simulink library "casper_library_correlator"  (Simulink 8.0)
settings: Solver=ode45  SolverMode=SingleTasking  StartTime=0.0  StopTime=10.0  RelTol=1e-3
values from neighbouring files (symbols this model uses):
  n_bits = eval(get_var('n_bits', 'defaults', defaults, varargin{:}))    [auto_tap_init.m]    (also in baseline_tap_init.m; bi_real_unscr_2x_init.m = get_var('n_bits', 'defaults', defaults, varargin{:}); bi_real_unscr_4x_init.m = get_var('n_bits', 'defaults', defaults, varargin{:}); bit_reverse_init.m = get_var('n_bits',varargin{:}))
libraries: xbsIndex_r4 x1360, casper_library_misc x140, casper_library_multipliers x32, xps_library x8, casper_library_delays x1, casper_library_correlator x1
(part 1 of 14)
settings Model: Creator=mdexter  LastModifiedBy=jmanley

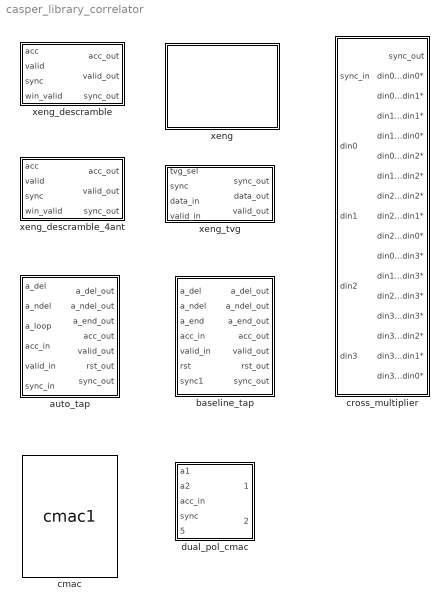
== system casper_library_correlator ==
  auto_tap : Subsystem  mask(auto_tap){n_ants=4, n_simultan=2, n_bits=4, acc_len=64, add_latency=1, mult_latency=2, bram_latency=2, mult_type=0, use_bram_delay=1}
      mask prompts: n_ants "Number of antennas (total inputs = n_ants*n_simultan below)"; n_simultan "Number of inputs fed-in simultaneously"; n_bits "Number of input bits (per complex component)"; acc_len "Accumulation length"; add_latency "Adder latency"; mult_latency "Multiplier latency"; bram_latency "BRAM latency"; mult_type "Multiplier Type (0=behavioural HDL, 1=embedded, 2=core)"; use_bram_delay "Implementation: Delay type (0=SLR, 1=BRAM)"
      mask init:
      | fix_pnt_pos = (n_bits-1)*2;
      | bit_growth = ceil(log2(acc_len));
      | ant_bits = ceil(log2(n_ants));
      | n_bits_out = (2*n_bits + 1 + bit_growth);
      | 
      | params = get_mask_params(gcb);
      | auto_tap_init(gcb, params{:});
      settings: AttributesFormatString=mult_typ=0, del_typ=1
  baseline_tap : Subsystem  mask(baseline_tap){n_ants=4, ant_sep=1, n_bits=4, acc_len=32, add_latency=1, mult_latency=2, bram_latency=2, mult_type=2, use_bram_delay=1}
      mask prompts: n_ants "Number of antennas"; ant_sep "Antenna Seperation"; n_bits "number of input bits (per complex component)"; acc_len "accumulation length"; add_latency "Adder latency"; mult_latency "Multiplier latency"; bram_latency "BRAM latency"; mult_type "Multiplier Type (0=behavioural HDL, 1=embedded, 2=core)"; use_bram_delay "Use BRAM delays"
      mask init:
      | fix_pnt_pos = (n_bits-1)*2;
      | bit_growth = ceil(log2(acc_len));
      | ant_bits = ceil(log2(n_ants));
      | n_bits_out = (2*n_bits + 1 + bit_growth);
      | 
      | params = get_mask_params(gcb);
      | baseline_tap_init(gcb, params{:});
      settings: AttributesFormatString=ant_sep=1, mult=2, bram=1
  cmac : casper_library_correlator/dual_pol_cmac/cmac1  Tag=cmac  acc_len=128  n_bits_a=4  bin_pt_a=3  n_bits_b=4  bin_pt_b=3  quantization=Truncate  overflow=Wrap  mult_latency=1  add_latency=1  in_latency=0  conv_latency=0  multiplier_implementation=embedded multiplier core
  cross_multiplier : Subsystem  mask(cross_multiplier){streams=4, aggregation=2, bit_width_in=4, binary_point_in=3, bit_width_out=9, binary_point_out=6, mult_latency=2, add_latency=1, overflow=Wrap, quantisation=Truncate, conv_latency=0}
      mask prompts: streams "Number input streams"; aggregation "Aggregation per stream"; bit_width_in "Bit width in"; binary_point_in "Binary point in"; bit_width_out "Bit width out"; binary_point_out "Binary point out"; mult_latency "Multiplier latency"; add_latency "Adder latency"; overflow "Overflow behaviour"; quantisation "Quantisation behaviour"; conv_latency "Bit width conversion latency"
      mask help: Cross multiplies aggregated complex input streams.
      mask init:
      | cross_multiplier_init(gcb, ...
      |     'streams', streams, ...
      |     'aggregation', aggregation, ...
      |     'bit_width_in', bit_width_in, ...
      |     'binary_point_in', binary_point_in, ...
      |     'bit_width_out', bit_width_out, ...
      |     'binary_point_out', binary_point_out, ...
      |     'mult_latency', mult_latency, ...
      |     'add_latency', add_latency, ...
      |     'overflow', overflow, ...
      |     'quantisation', quantisation, ...
      |     'conv_latency', conv_latency);
      mask TypeOptions overflow: Wrap | Saturate | Error
      mask TypeOptions quantisation: Truncate | Round  (unbiased: +/- Inf) | Round  (unbiased: even values)
  dual_pol_cmac : Subsystem  AncestorBlock=casper_library_correlator/dual_pol_cmac  mask{acc_len=128, n_bits_in=4, bin_pt_in=3, mult_latency=1, add_latency=1, multiplier_implementation=embedded multiplier core}
      mask prompts: acc_len "Number of accumulations"; n_bits_in "Number of bits in"; bin_pt_in "Binary point in"; mult_latency "Multiplier latency"; add_latency "Adder latency"; multiplier_implementation "Multiplier implementation"
      mask init:
      | bit_growth = ceil(log2(acc_len));
      | n_bits_out = (n_bits_in*2 + 1 + bit_growth);
      | bin_pt_out=(bin_pt_in*2);
      | 
      | cmacs = find_system(gcb, 'lookUnderMasks', 'all', 'FollowLinks','on','tag', 'cmac');
      | for i=1:length(cmacs),
      |     reuse_block(get_param(cmacs{i},'Parent'),get_param(cmacs{i},'Name'),'casper_library_correlator/cmac',...
      |             'mult_latency',num2str(mult_latency),...            
      |             'add_latency',num2str(add_latency),...
      |             'acc_len',num2str(acc_len),...
      |             'n_bits_a',num2str(n_bits_in),...
      |             'n_bits_b',num2str(n_bits_in),...
      |             'bin_pt_a',num2str(n_bits_in-1),...
      |             'bin_pt_b',num2str(n_bits_in-1),...
      |             'multiplier_implementation',multiplier_implementation,...
      |             'LinkStatus','inactive');
      | end
      mask TypeOptions multiplier_implementation: behavioral HDL | standard core | embedded multiplier core
  xeng : Subsystem  Tag=casper:xeng  mask(xeng){n_ants=0, n_bits=4, acc_len=128, demux_factor=4, add_latency=1, mult_latency=1, bram_latency=2, use_ded_mult=1, use_bram_delay=1}
      mask prompts: n_ants "Number of antennas"; n_bits "Bit-width of samples in"; acc_len "Accumulation length"; add_latency "Adder latency"; mult_latency "Multiplier latency"; bram_latency "BRAM latency"; use_ded_mult "Implementation: Multiplier type (0=slices 1=embedded 2=bram)"; use_bram_delay "Implementation: Delay type (0=SLR, 1=BRAM)"
      mask help: CASPER X engine with added internal valid data masking functionality, descramble and integral demux. Based on Aaron Parsons' and Lynn Urry's original X engine design.
      mask init:
      | xeng_init(gcb, ...
      |     'n_ants', n_ants, ...
      |     'n_bits', n_bits, ...
      |     'acc_len', acc_len, ...
      |     'demux_factor', demux_factor, ...
      |     'add_latency', add_latency, ...
      |     'mult_latency', mult_latency, ...
      |     'bram_latency', bram_latency, ...
      |     'use_ded_mult', use_ded_mult, ...
      |     'use_bram_delay', use_bram_delay);
      mask TypeOptions demux_factor: 1 | 2 | 4 | 8
  xeng_descramble : Subsystem  mask(xeng_descramble){num_ants=8, n_bits=4, acc_len=128, demux_factor=8}
      mask prompts: num_ants "Number of Antennas"; n_bits "Input Bitwidth"; acc_len "X engine accumulation length"; demux_factor "Demux Factor"
      mask help:
      | NOT TESTED FOR non-2^N antennas.
      |
      | Descrambles X engine output. Optionally demuxes output.
      mask init:
      | num_taps = floor(num_ants/2) + 1;
      | ant_bits = ceil(log2(num_ants));
      | num_validins = num_ants*num_taps;
      | validin_bits = floor(log2(num_validins))+1;
      | demux_bits = floor(log2(demux_factor))+1;
      | acc_len_bits = floor(log2(acc_len))+1;
      | num_ants_bits = floor(log2(num_ants))+1;
      | taps_bits = floor(log2(num_taps))+1;
      | pivot_pnt = num_ants/2*(num_taps) + num_taps*num_ants/4;
      | num_elements = nchoosek(num_ants, 2) + num_ants;
      | elements_bits = floor(log2(num_elements)) + 1;
      | n_bits_xeng_out = (2*n_bits + acc_len_bits);
      | n_bits_in = 2^(ceil(log2(n_bits_xeng_out)))*8;
      | 
      | ship_el_del = floor(acc_len*num_ants/num_validins/demux_factor) - 1;
      | 
      | if (ship_el_del < 0)
      |     errordlg('Insufficient output space for this configuration. Try a lower demux setting. Else you need fewer antennas or longer xeng acc time.');
      |     ship_el_del=0;
      | end
      | 
      | if (ship_el_del == 0)
      |     ship_el_cnt = demux_factor*num_elements-1;
      |     %in this case we're outputting multiple words back-to-back.
      | else
      |     ship_el_cnt = demux_factor*num_elements;
      |     %in this case we're outputting one word at a time.
      | end
      | 
      | ship_el_del_bits = ceil(log2(ship_el_del + 1));
      | 
      | if (ship_el_del_bits == 0)
      |     ship_el_del_bits =1;
      | end
      | 
      | fmtstr = sprintf('num_ants=%d',num_ants);
      | set_param(gcb, 'AttributesFormatString', fmtstr);
      settings: AttributesFormatString=num_ants=8
  xeng_descramble_4ant : Subsystem  mask(xeng_descramble){n_bits=4, acc_len=128, demux_factor=8}
      mask prompts: n_bits "Input Bitwidth"; acc_len "X engine accumulation length"; demux_factor "Demux Factor"
      mask help:
      | NOT TESTED FOR non-2^N antennas.
      |
      | Descrambles X engine output. Optionally demuxes output.
      mask init:
      | num_ants=4;
      | num_taps = floor(num_ants/2) + 1;
      | ant_bits = ceil(log2(num_ants));
      | num_validins = num_ants*num_taps;
      | validin_bits = floor(log2(num_validins))+1;
      | demux_bits = floor(log2(demux_factor))+1;
      | acc_len_bits = floor(log2(acc_len))+1;
      | num_ants_bits = floor(log2(num_ants))+1;
      | taps_bits = floor(log2(num_taps))+1;
      | pivot_pnt = num_ants/2*(num_taps) + num_taps*num_ants/4;
      | num_elements = nchoosek(num_ants, 2) + num_ants;
      | elements_bits = floor(log2(num_elements)) + 1;
      | n_bits_xeng_out = (2*n_bits + acc_len_bits);
      | n_bits_in = 2^(ceil(log2(n_bits_xeng_out)))*8;
      | 
      | ship_el_del = floor(acc_len*num_ants/num_validins/demux_factor) - 1;
      | 
      | if (ship_el_del < 0)
      |     errordlg('Insufficient output space for this configuration. Try a lower demux setting. Else you need fewer antennas or longer xeng acc time.');
      |     ship_el_del=0;
      | end
      | 
      | if (ship_el_del == 0)
      |     ship_el_cnt = demux_factor*num_elements-1;
      |     %in this case we're outputting multiple words back-to-back.
      | else
      |     ship_el_cnt = demux_factor*num_elements;
      |     %in this case we're outputting one word at a time.
      | end
      | 
      | ship_el_del_bits = ceil(log2(ship_el_del + 1));
      | 
      | if (ship_el_del_bits == 0)
      |     ship_el_del_bits =1;
      | end
      | 
      | fmtstr = sprintf('num_ants=%d',num_ants);
      | set_param(gcb, 'AttributesFormatString', fmtstr);
      settings: AttributesFormatString=num_ants=4
  xeng_tvg : Subsystem  mask{ant_bits=2, x_int_bits=5, sync_period=15}
      mask prompts: ant_bits "Number of Antennas (2^?):"; x_int_bits "X Integration Length (2^?):"; sync_period "Sync Pulse Period (2^?):"

== system casper_library_correlator/auto_tap ==
  a_del : Inport
  a_ndel : Inport  Port=2
  a_loop : Inport  Port=3
  acc_in : Inport  Port=4
  valid_in : Inport  Port=5
  sync_in : Inport  Port=6
  delay : Subsystem  AncestorBlock=casper_library_delays/delay_bram  mask(delay_bram){DelayLen=126, bram_latency=2, use_dsp48=off, async=off}
      mask prompts: DelayLen "Delay By:"; bram_latency "BRAM Latency"; use_dsp48 "Use DSP48"; async "asynchronous operation"
      mask help: A delay block that uses BRAM for its storage.
      mask init:
      | delay_bram_init(gcb, ...
      |     'DelayLen', DelayLen, ...
      |     'bram_latency', bram_latency, ...
      |     'use_dsp48', use_dsp48, ...
      |     'async', async);
      mask Help: eval('xlWeb(''http://casper.berkeley.edu/wiki/Delay_bram'')')
  dual_pol_cmac : Subsystem  AncestorBlock=casper_library_correlator/dual_pol_cmac  mask{acc_len=128, n_bits_in=4, bin_pt_in=3, mult_latency=1, add_latency=1, multiplier_implementation=embedded multiplier core}
      mask prompts: acc_len "Number of accumulations"; n_bits_in "Number of bits in"; bin_pt_in "Binary point in"; mult_latency "Multiplier latency"; add_latency "Adder latency"; multiplier_implementation "Multiplier implementation"
      mask init: same as casper_library_correlator/dual_pol_cmac
      mask TypeOptions multiplier_implementation: behavioral HDL | standard core | embedded multiplier core
  sync_delay : casper_library_delays/sync_delay  DelayLen=71
  a_del_out : Outport
  a_ndel_out : Outport  Port=2
  a_end_out : Outport  Port=3
  acc_out : Outport  Port=4
  valid_out : Outport  Port=5
  rst_out : Outport  Port=6
  sync_out : Outport  Port=7
  wires:
  sync_in/1 -> sync_delay/1, dual_pol_cmac/4(sync), rst_out/1
  a_del/1 -> dual_pol_cmac/1(a1), a_del_out/1
  dual_pol_cmac/1(acc_out) -> acc_out/1
  acc_in/1 -> dual_pol_cmac/3(acc_in)
  dual_pol_cmac/2(valid_out) -> valid_out/1
  valid_in/1 -> dual_pol_cmac/5(valid_in)
  a_ndel/1 -> dual_pol_cmac/2(a2), a_ndel_out/1
  a_loop/1 -> delay/1(din)
  delay/1(dout) -> a_end_out/1
  sync_delay/1 -> sync_out/1

== system casper_library_correlator/baseline_tap ==
  a_del : Inport
  a_ndel : Inport  Port=2
  a_end : Inport  Port=3
  acc_in : Inport  Port=4
  valid_in : Inport  Port=5
  rst : Inport  Port=6
  sync1 : Inport  Port=7
  Constant : xbsIndex_r4/Constant  const=ant_sep * acc_len  gui_display_data_type=Fixed-point  arith_type=Unsigned  n_bits=ant_bits + bit_growth  bin_pt=0  preci_type=Single  exp_width=8  frac_width=24  explicit_period=on  period=1  equ=P=C  opselect=C  inp2=PCIN>>17  opr=+  inp1=P  carry=CIN  dbl_ovrd=off  block_type=constant
      settings: block_version=9.1.01
  Convert : xbsIndex_r4/Convert  gui_display_data_type=Fixed-point  arith_type=Unsigned  n_bits=1  bin_pt=0  float_type=Single  exp_bits=8  fraction_bits=24  quantization=Truncate  overflow=Wrap  en=off  latency=0  dbl_ovrd=off  pipeline=off  block_type=convert
      settings: xl_area=[0, 0, 0, 0, 0, 0, 0]
  Counter : xbsIndex_r4/Counter  cnt_type=Count Limited  cnt_to=n_ants * acc_len - 1  operation=Up  start_count=0  cnt_by_val=1  arith_type=Unsigned  n_bits=ant_bits + bit_growth  bin_pt=0  load_pin=off  rst=on  en=off  explicit_period=off  period=1  dbl_ovrd=off  use_behavioral_HDL=off  implementation=Fabric  use_rpm=on  block_type=counter
      settings: xl_area=[0, 0, 0, 0, 0, 0, 0]  block_version=9.1.01
  Delay{1,3,7..8} (4 alike) : xbsIndex_r4/Delay  rst=off  infoeditControl=Selection of Reset will increase slice count due to use of real FFs and instead of SRLs  en=off  latency=1  dbl_ovrd=off  reg_retiming=on  block_type=delay
      settings: xl_area=[0, 0, 0, 0, 0, 0, 0]  block_version=9.1.01
  Mux : xbsIndex_r4/Mux  inputs=2  en=off  latency=1  precision=Full  arith_type="Signed  (2's comp)"  n_bits=8  bin_pt=2  quantization=Truncate  overflow=Wrap  dbl_ovrd=off  block_type=mux
      settings: xl_area=[0, 0, 0, 0, 0, 0, 0]  block_version=9.1.01
  Relational : xbsIndex_r4/Relational  mode=a<b  en=off  latency=0  dbl_ovrd=off  block_type=relational
      settings: xl_area=[0, 0, 0, 0, 0, 0, 0]  block_version=9.1.01
  delay : Subsystem  AncestorBlock=casper_library_delays/delay_bram  mask(delay_bram){DelayLen=acc_len, bram_latency=bram_latency, use_dsp48=off, async=off}
      mask prompts: DelayLen "Delay By:"; bram_latency "BRAM Latency"; use_dsp48 "Use DSP48"; async "asynchronous operation"
      mask help: A delay block that uses BRAM for its storage.
      mask init:
      | delay_bram_init(gcb, ...
      |     'DelayLen', DelayLen, ...
      |     'bram_latency', bram_latency, ...
      |     'use_dsp48', use_dsp48, ...
      |     'async', async);
      mask Help: eval('xlWeb(''http://casper.berkeley.edu/wiki/Delay_bram'')')
  dual_pol_cmac : Subsystem  AncestorBlock=casper_library_correlator/dual_pol_cmac  mask{acc_len=128, n_bits_in=4, bin_pt_in=3, mult_latency=1, add_latency=1, multiplier_implementation=embedded multiplier core}
      mask prompts: acc_len "Number of accumulations"; n_bits_in "Number of bits in"; bin_pt_in "Binary point in"; mult_latency "Multiplier latency"; add_latency "Adder latency"; multiplier_implementation "Multiplier implementation"
      mask init: same as casper_library_correlator/dual_pol_cmac
      mask TypeOptions multiplier_implementation: behavioral HDL | standard core | embedded multiplier core
  a_del_out : Outport
  a_ndel_out : Outport  Port=2
  a_end_out : Outport  Port=3
  acc_out : Outport  Port=4
  valid_out : Outport  Port=5
  rst_out : Outport  Port=6
  sync_out : Outport  Port=7
  wires:
  sync1/1 -> sync_out/1
  Delay1/1 -> dual_pol_cmac/4(sync), rst_out/1
  Delay8/1 -> a_end_out/1
  Delay7/1 -> a_ndel_out/1
  Delay3/1 -> dual_pol_cmac/1(a1), a_del_out/1
  a_end/1 -> Delay8/1, Mux/3
  a_ndel/1 -> Delay7/1, Mux/2
  valid_in/1 -> dual_pol_cmac/5(valid_in)
  dual_pol_cmac/2(valid_out) -> valid_out/1
  acc_in/1 -> dual_pol_cmac/3(acc_in)
  dual_pol_cmac/1(acc_out) -> acc_out/1
  a_del/1 -> delay/1(din)
  rst/1 -> Counter/1, Delay1/1
  Convert/1 -> Mux/1
  Relational/1 -> Convert/1
  Constant/1 -> Relational/2
  Counter/1 -> Relational/1
  Mux/1 -> dual_pol_cmac/2(a2)
  delay/1(dout) -> Delay3/1
